simulink model "SensorlessStartup"  (R2026b)
settings: Solver=VariableStepAuto
undefined symbols (not defined in the file or in its folder): startupCfg
settings Model: Creator=24322  LastModifiedBy=24322

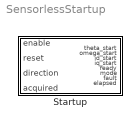
== system SensorlessStartup ==
  Startup : Subsystem  mask{startupCfg=startupCfg}
      mask prompts: startupCfg "Startup configuration"

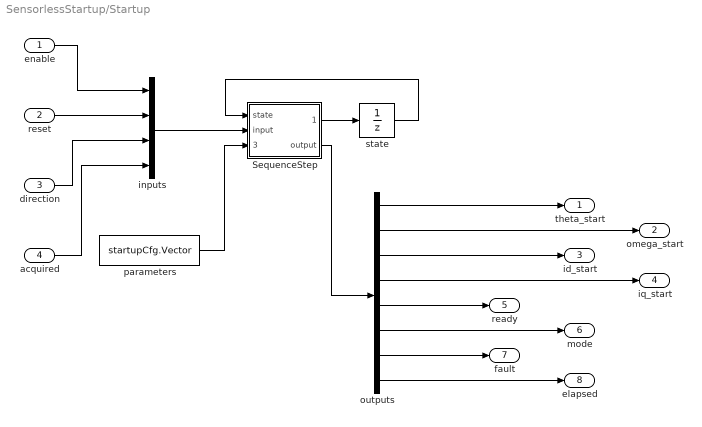
== system SensorlessStartup/Startup ==
  enable : Inport  SampleTime=startupCfg.Ts
  reset : Inport  Port=2  SampleTime=startupCfg.Ts
  direction : Inport  Port=3  SampleTime=startupCfg.Ts
  acquired : Inport  Port=4  SampleTime=startupCfg.Ts
  SequenceStep : MATLAB Function  TreatAsAtomicUnit=on
  inputs : Mux
  outputs : Demux  Outputs=8
  parameters : Constant  Value=startupCfg.Vector
  state : UnitDelay  InitialCondition=startupCfg.State0  SampleTime=startupCfg.Ts
  theta_start : Outport
  omega_start : Outport  Port=2
  id_start : Outport  Port=3
  iq_start : Outport  Port=4
  ready : Outport  Port=5
  mode : Outport  Port=6
  fault : Outport  Port=7
  elapsed : Outport  Port=8
  wires:
  outputs/8 -> elapsed/1
  outputs/7 -> fault/1
  outputs/6 -> mode/1
  outputs/5 -> ready/1
  outputs/4 -> iq_start/1
  outputs/3 -> id_start/1
  outputs/2 -> omega_start/1
  outputs/1 -> theta_start/1
  acquired/1 -> inputs/4
  direction/1 -> inputs/3
  reset/1 -> inputs/2
  enable/1 -> inputs/1
  SequenceStep/2(output) -> outputs/1
  SequenceStep/1(nextState) -> state/1
  parameters/1 -> SequenceStep/3(parameter)
  inputs/1 -> SequenceStep/2(input)
  state/1 -> SequenceStep/1(state)

== matlab function SensorlessStartup/Startup/SequenceStep ==
  data: state input; nextState output; input input; parameter input; output output
function [nextState,output]=startup_step(state,input,parameter)
%#codegen
%STARTUP_STEP Stateless sequencing; Unit Delay owns [mode,n,theta,ifN,fault].
% input = [enable;reset;direction;acquired]. Angles are software field angles.
parameter=cast(parameter,'like',state);
nextState=state;output=zeros(8,1,'like',state);
sampleTime=parameter(1);theta=state(3);mode=state(1);count=state(2);
omega=cast(0,'like',state);id=omega;ready=omega;fault=state(5);
if input(1)<0.5 || input(2)>0.5
    nextState(:)=0;nextState(3)=parameter(2);output(1)=parameter(2);
    return
end
if mode==7
    output(1)=theta;output(6)=7;output(7)=fault;output(8)=count*sampleTime;
    return
end
direction=cast(input(3),'like',state);
if abs(direction)~=1
    nextState(1)=7;nextState(2)=0;nextState(5)=2;
    output(1)=theta;output(6)=7;output(7)=2;
    return
end
if input(4)>0.5
    nextState(1)=6;nextState(2)=0;nextState(5)=0;
    output(1)=theta;output(6)=6;
    return
end
nextState(2)=count+1;
if mode==0
    nextState(1)=1;nextState(2)=0;
elseif mode==1
    if count+1>=parameter(6),nextState(1)=2;nextState(2)=0;end
elseif mode==2
    theta=-direction*pi/2;
    id=parameter(3)*min(count/parameter(8),1);
    if count+1>=parameter(7),nextState(1)=3;nextState(2)=0;end
elseif mode==3
    theta=-direction*pi/2*(1-min(count/parameter(10),1));
    id=parameter(3);
    if count<parameter(10),omega=direction*pi/(2*sampleTime*parameter(10));end
    if count+1>=parameter(9)
        nextState(1)=4;nextState(2)=0;nextState(4)=0;
    end
elseif mode==4 || mode==5
    if mode==4
        omega=direction*parameter(5)*min(count/parameter(11),1);
        id=parameter(3)+(parameter(4)-parameter(3))*min(count/parameter(12),1);
        if count+1>=parameter(11),nextState(1)=5;nextState(2)=0;end
    else
        omega=direction*parameter(5);id=parameter(4);
    end
    ready=cast(abs(omega)>=parameter(14),'like',state);
    nextState(4)=state(4)+1;
    if nextState(4)>=parameter(13)
        nextState(1)=7;nextState(2)=0;nextState(5)=1;
    end
elseif mode==6
    nextState(2)=0;
else
    nextState(1)=7;nextState(2)=0;nextState(5)=3;
end
if mode==4 || mode==5
    nextTheta=theta+sampleTime*omega;
    nextState(3)=atan2(sin(nextTheta),cos(nextTheta));
else
    nextState(3)=theta;
end
output(1)=theta;output(2)=omega;output(3)=id;output(4)=0;
output(5)=ready;output(6)=mode;output(7)=fault;output(8)=count*sampleTime;
end
